simulink library "Lib_Piccolo"  (R2018b)
settings: Solver=VariableStepAuto  StartTime=0.0  StopTime=10.0  RelTol=1e-3
values from neighbouring files (symbols this model uses):
  AccelErrInt2Brakes = 0.15    [SimulationControlConfig16P.m]    (also in SimulationControlConfig16P_LEGACY.m; SimulationControlConfigTAILLESS.m = 0.2; SimulationControlConfigUTAIL.m = 0.2)
  AileronMax = 25    [SimulationControlConfig16P.m]    (also in SimulationControlConfig16P_LEGACY.m; SimulationControlConfigTAILLESS.m; SimulationControlConfigUTAIL.m)
  AileronPower = 0.00268    [SimulationControlConfig16P.m]    (also in SimulationControlConfig16P_LEGACY.m; SimulationControlConfigTAILLESS.m; SimulationControlConfigUTAIL.m)
  AileronSurfaceMax = 45    [SimulationControlConfig16P.m]    (also in SimulationControlConfig16P_LEGACY.m)
  AileronTrim = 0    [SimulationControlConfig16P.m]    (also in SimulationControlConfig16P_LEGACY.m; SimulationControlConfigTAILLESS.m; SimulationControlConfigUTAIL.m)
  Alt = 1000 + TerrainHeight    [SimulationStateConfig.m]
  AltCruise_m = testPlans(testIndx).terrainElevation * 0.3048 + 200    [SimulationControlConfig16P.m]    (also in SimulationControlConfigTAILLESS.m = 1083; SimulationControlConfigUTAIL.m = testPlans(testIndx).terrainElevation * 0.3048 + 152)
  AltitudeRate2PitchCmdIntegratorInit = 0.1    [SimulationControlPre.m]
  AltMax = 10000    [SimulationControlConfig16P.m]    (also in SimulationControlConfig16P_LEGACY.m; SimulationControlConfigTAILLESS.m; SimulationControlConfigUTAIL.m)
  AltMaxAccel = 1.25    [SimulationControlConfig16P.m]    (also in SimulationControlConfig16P_LEGACY.m = 0.9; SimulationControlConfigTAILLESS.m = 1.7; SimulationControlConfigUTAIL.m = 2)
  AltMin = 0    [SimulationControlConfig16P.m]    (also in SimulationControlConfig16P_LEGACY.m; SimulationControlConfigTAILLESS.m; SimulationControlConfigUTAIL.m)
  AltRateCmd2Pitch = 0.50    (= 0.5)    [SimulationControlConfig16P.m]    (also in SimulationControlConfig16P_LEGACY.m = 0.6; SimulationControlConfigTAILLESS.m = 0.2; SimulationControlConfigUTAIL.m = 0.3)
  AltRateError2Pitch = 0.40    (= 0.4)    [SimulationControlConfig16P.m]    (also in SimulationControlConfig16P_LEGACY.m; SimulationControlConfigTAILLESS.m = 0.55; SimulationControlConfigUTAIL.m = 0.55)
  AltRateErrorInt2Pitch = 0.50    (= 0.5)    [SimulationControlConfig16P.m]    (also in SimulationControlConfig16P_LEGACY.m = 0.45; SimulationControlConfigTAILLESS.m; SimulationControlConfigUTAIL.m = 0.75)
  AltRateLpfCutOff = 3    [SimulationControlConfig16P.m]    (also in SimulationControlConfig16P_LEGACY.m; SimulationControlConfigTAILLESS.m = 2; SimulationControlConfigUTAIL.m = 2)
  AutoNosegear2Rudder = 26    [SimulationControlConfig16P.m]    (also in SimulationControlConfig16P_LEGACY.m; SimulationControlConfigTAILLESS.m = 25.2; SimulationControlConfigUTAIL.m = 14)
  b = 5.54    [SimulationControlConfig16P.m]    (also in SimulationControlConfig16P_LEGACY.m; SimulationControlConfigTAILLESS.m = 2.37; SimulationControlConfigUTAIL.m = 2.37)
  Bank2AileronIntegratorInit = 0    [SimulationControlPre.m]
  BankMax_User = BankMax_User/180*pi    (= 0.523598775598)    [SimulationControlConfig16P.m]    (also in SimulationControlConfig16P_LEGACY.m; SimulationControlConfigTAILLESS.m = 0.610865238198; SimulationControlConfigUTAIL.m = 0.628318530718)
  baseLegFlaps = 20    [SimulationControlConfig16P.m]    (also in SimulationControlConfig16P_LEGACY.m = 0; SimulationControlConfigTAILLESS.m = 15; SimulationControlConfigUTAIL.m = 10)
  C = GeneticOpt.C    [SimulationCostFunction.m]
  c = Sw/b    (= 0.841696750903)    [SimulationControlConfig16P.m]    (also in SimulationControlConfig16P_LEGACY.m; SimulationControlConfigTAILLESS.m = 0.354008438819; SimulationControlConfigUTAIL.m = 0.354008438819)
  cell2WheelFactorMG = 5.98    [SimulationSensorConfig16P_LEGACY.m]
  cell2WheelFactorNG = 1    [SimulationSensorConfig16P_LEGACY.m]
  cellSatMaxMG = 15000    [SimulationSensorConfig16P.m]    (also in SimulationSensorConfig16P_LEGACY.m; SimulationSensorConfigTAILLESS7P.m; SimulationSensorConfigUTAIL7P.m)
  cellSatMaxNG = 1000    [SimulationSensorConfig16P.m]    (also in SimulationSensorConfig16P_LEGACY.m; SimulationSensorConfigTAILLESS7P.m; SimulationSensorConfigUTAIL7P.m)
  cellSatMinMG = -15000    [SimulationSensorConfig16P.m]    (also in SimulationSensorConfig16P_LEGACY.m; SimulationSensorConfigTAILLESS7P.m; SimulationSensorConfigUTAIL7P.m)
  cellSatMinNG = -1000    [SimulationSensorConfig16P.m]    (also in SimulationSensorConfig16P_LEGACY.m; SimulationSensorConfigTAILLESS7P.m; SimulationSensorConfigUTAIL7P.m)
  CL_Limit = CL_Max    (= 0.54)    [SimulationControlConfig16P.m]    (also in SimulationControlConfig16P_LEGACY.m; SimulationControlConfigTAILLESS.m; SimulationControlConfigUTAIL.m = 0.53)
  CL_Max = 0.54    [SimulationControlConfig16P.m]    (also in SimulationControlConfig16P_LEGACY.m; SimulationControlConfigTAILLESS.m; SimulationControlConfigUTAIL.m = 0.53)
  CL_Max_Nom = 0.465    [SimulationControlConfig16P.m]    (also in SimulationControlConfig16P_LEGACY.m; SimulationControlConfigTAILLESS.m = 0.39; SimulationControlConfigUTAIL.m)
  CL_Min = 0    [SimulationControlConfig16P.m]    (also in SimulationControlConfig16P_LEGACY.m; SimulationControlConfigTAILLESS.m; SimulationControlConfigUTAIL.m)
  ClimbMaxFraction = 0.35    [SimulationControlConfig16P.m]    (also in SimulationControlConfig16P_LEGACY.m = 0.24; SimulationControlConfigTAILLESS.m = 0.19; SimulationControlConfigUTAIL.m = 0.21)
  ClimboutMaxBank = 7.0    (= 7)    [SimulationControlConfig16P.m]    (also in SimulationControlConfig16P_LEGACY.m; SimulationControlConfigTAILLESS.m = 5; SimulationControlConfigUTAIL.m)
  ClimboutTimer = 7.0    (= 7)    [SimulationControlConfig16P.m]    (also in SimulationControlConfig16P_LEGACY.m; SimulationControlConfigTAILLESS.m; SimulationControlConfigUTAIL.m)
  dCl_per_dFlap = 0.005581818    [SimulationControlConfig16P.m]    (also in SimulationControlConfig16P_LEGACY.m = 0; SimulationControlConfigTAILLESS.m = 0; SimulationControlConfigUTAIL.m = 0)
  DecelerationCmd = 3.1    [SimulationControlConfig16P.m]    (also in SimulationControlConfig16P_LEGACY.m; SimulationControlConfigTAILLESS.m = 0.1; SimulationControlConfigUTAIL.m = 0.1)
  DeRotateLogicEndTimer = abs((NoseDownLimit_Deg-1)/DeRotateRamp_Dps)    [SimulationControlConfig16P.m]    (also in SimulationControlConfig16P_LEGACY.m; SimulationControlConfigTAILLESS.m; SimulationControlConfigUTAIL.m)
  DeRotateLogicHoldNoseUpTimer = 0.1    [SimulationControlConfig16P.m]    (also in SimulationControlConfig16P_LEGACY.m; SimulationControlConfigTAILLESS.m; SimulationControlConfigUTAIL.m)
  DeRotateLogicTimerTimeout = 2    [SimulationControlConfig16P.m]    (also in SimulationControlConfig16P_LEGACY.m; SimulationControlConfigTAILLESS.m; SimulationControlConfigUTAIL.m)
  DeRotateLowerCmdSaturation = 0    [SimulationControlConfig16P.m]    (also in SimulationControlConfig16P_LEGACY.m; SimulationControlConfigTAILLESS.m; SimulationControlConfigUTAIL.m)
  DeRotateRamp_Dps = 3    [SimulationControlConfig16P.m]    (also in SimulationControlConfig16P_LEGACY.m; SimulationControlConfigTAILLESS.m = 8; SimulationControlConfigUTAIL.m = 8)
  DeRotateUpperCmdSaturation = 7    [SimulationControlConfig16P.m]    (also in SimulationControlConfig16P_LEGACY.m; SimulationControlConfigTAILLESS.m; SimulationControlConfigUTAIL.m)
  DescentMaxFraction = 0.22    [SimulationControlConfig16P.m]    (also in SimulationControlConfig16P_LEGACY.m = 0.2; SimulationControlConfigTAILLESS.m = 0.17; SimulationControlConfigUTAIL.m = 0.17)
  DesktopSimTerrainOffset_m = 0.406    [SimulationAircraftConfig.m]
  downwindFlaps = 0    [SimulationControlConfig16P.m]    (also in SimulationControlConfig16P_LEGACY.m; SimulationControlConfigTAILLESS.m; SimulationControlConfigUTAIL.m)
  DP_init = 0.5*1.225*V_init^2    [SimulationControlConfig16P.m]    (also in SimulationControlConfig16P_LEGACY.m; SimulationControlConfigTAILLESS.m; SimulationControlConfigUTAIL.m)
  dscNoiseMG = 1    [SimulationSensorConfig16P_LEGACY.m]
  dscNoiseNG = 0.25    [SimulationSensorConfig16P_LEGACY.m]
  DSCnumBits = 24    [SimulationSensorConfig16P.m]    (also in SimulationSensorConfig16P_LEGACY.m; SimulationSensorConfigTAILLESS7P.m; SimulationSensorConfigUTAIL7P.m)
  DSCRangeMaxMG = 15000    [SimulationSensorConfig16P.m]    (also in SimulationSensorConfig16P_LEGACY.m; SimulationSensorConfigTAILLESS7P.m; SimulationSensorConfigUTAIL7P.m)
  DSCRangeMaxNG = 1000    [SimulationSensorConfig16P.m]    (also in SimulationSensorConfig16P_LEGACY.m; SimulationSensorConfigTAILLESS7P.m; SimulationSensorConfigUTAIL7P.m)
  DSCRangeMinMG = -15000    [SimulationSensorConfig16P.m]    (also in SimulationSensorConfig16P_LEGACY.m; SimulationSensorConfigTAILLESS7P.m; SimulationSensorConfigUTAIL7P.m)
  DSCRangeMinNG = -1000    [SimulationSensorConfig16P.m]    (also in SimulationSensorConfig16P_LEGACY.m; SimulationSensorConfigTAILLESS7P.m; SimulationSensorConfigUTAIL7P.m)
  dt = DLLSim.dt    [SimulationTimeStep.m]    (also in SimulationTrim.m = 0.02)
  EarlyTouchdownThreshold = 3.0    (= 3)    [SimulationControlConfig16P.m]    (also in SimulationControlConfig16P_LEGACY.m; SimulationControlConfigTAILLESS.m = 2.2; SimulationControlConfigUTAIL.m = 2.5)
  ElevatorDeflectionRate = 15    [SimulationControlConfig16P.m]    (also in SimulationControlConfig16P_LEGACY.m = 12; SimulationControlConfigTAILLESS.m = 10; SimulationControlConfigUTAIL.m = 12)
  ElevatorMax = 25    [SimulationControlConfig16P.m]    (also in SimulationControlConfig16P_LEGACY.m; SimulationControlConfigTAILLESS.m; SimulationControlConfigUTAIL.m)
  ElevatorPower = -0.002209    [SimulationControlConfig16P.m]    (also in SimulationControlConfig16P_LEGACY.m; SimulationControlConfigTAILLESS.m = -0.002956; SimulationControlConfigUTAIL.m = -0.00205983)
  ElevatorTrim = -3.5    [SimulationControlConfig16P.m]    (also in SimulationControlConfig16P_LEGACY.m; SimulationControlConfigTAILLESS.m = -6; SimulationControlConfigUTAIL.m = -8)
  elevonBias = 0    [SimulationControlConfig16P.m]    (also in SimulationControlConfig16P_LEGACY.m; SimulationControlConfigTAILLESS.m; SimulationControlConfigUTAIL.m)
  Enable_TAS_Protection = 0    [SimulationControlConfig16P.m]    (also in SimulationControlConfig16P_LEGACY.m; SimulationControlConfigTAILLESS.m; SimulationControlConfigUTAIL.m)
  EnableCrossTrackAbort = 1    [SimulationControlConfig16P.m]    (also in SimulationControlConfigTAILLESS.m; SimulationControlConfigUTAIL.m)
  EnergyBandwidth = 0.02    [SimulationControlConfig16P.m]    (also in SimulationControlConfig16P_LEGACY.m; SimulationControlConfigTAILLESS.m = 0.06; SimulationControlConfigUTAIL.m = 0.06)
  EngineLhFuelCut = 0    [SimulationAircraftConfig.m]
  EngineRhFuelCut = 0    [SimulationAircraftConfig.m]
  FastThrottleRate = 0.075    [SimulationControlConfig16P.m]    (also in SimulationControlConfig16P_LEGACY.m = 0.05; SimulationControlConfigTAILLESS.m = 0.1; SimulationControlConfigUTAIL.m = 0.1)
  FilterWarmUpTime = 2    [SimulationSensorConfig16P.m]    (also in SimulationSensorConfig16P_LEGACY.m; SimulationSensorConfigTAILLESS7P.m; SimulationSensorConfigUTAIL7P.m)
  finalApproachFlaps = 20    [SimulationControlConfig16P.m]    (also in SimulationControlConfig16P_LEGACY.m = 0; SimulationControlConfigTAILLESS.m = 22; SimulationControlConfigUTAIL.m = 10)
  FinalDescentSlope_Deg = testPlans(testIndx).descentSlope    [SimulationControlConfig16P.m]    (also in SimulationControlConfig16P_LEGACY.m; SimulationControlConfigTAILLESS.m; SimulationControlConfigUTAIL.m)
  flapMax = 0    [SimulationControlConfig16P.m]    (also in SimulationControlConfig16P_LEGACY.m; SimulationControlConfigTAILLESS.m; SimulationControlConfigUTAIL.m)
  flapRate = 7.5    [SimulationControlConfig16P.m]    (also in SimulationControlConfig16P_LEGACY.m; SimulationControlConfigTAILLESS.m = 6.6; SimulationControlConfigUTAIL.m)
  FlareHeight = 5    [SimulationControlConfig16P.m]    (also in SimulationControlConfig16P_LEGACY.m = 4.8; SimulationControlConfigTAILLESS.m = 2.5; SimulationControlConfigUTAIL.m = 2)
  FlareVerticalRate_mps = -0.4    [SimulationControlConfig16P.m]    (also in SimulationControlConfig16P_LEGACY.m = -0.5; SimulationControlConfigTAILLESS.m = -0.15; SimulationControlConfigUTAIL.m = -0.15)
  Fp_Aileron = 0.55*2*pi*RollRateLpfCutoff*dt    [SimulationControlConfig16P.m]    (also in SimulationControlConfig16P_LEGACY.m; SimulationControlConfigTAILLESS.m; SimulationControlConfigUTAIL.m)
  Fp_Alt = 0.55*AltBandwidth    (= 0.099)    [SimulationControlConfig16P.m]    (also in SimulationControlConfig16P_LEGACY.m; SimulationControlConfigTAILLESS.m = 0.587477826221; SimulationControlConfigUTAIL.m = 0.69115038379)
  Fp_AltRate = 0.55*2*pi*AltRateLpfCutOff*dt    [SimulationControlConfig16P.m]    (also in SimulationControlConfig16P_LEGACY.m; SimulationControlConfigTAILLESS.m; SimulationControlConfigUTAIL.m)
  Fp_Elevator = 0.55*2*pi*PitchRateLpfCutoff*dt    [SimulationControlConfig16P.m]    (also in SimulationControlConfig16P_LEGACY.m; SimulationControlConfigTAILLESS.m; SimulationControlConfigUTAIL.m)
  Fp_Energy = 0.55*2*pi*EnergyBandwidth    (= 0.069115038379)    [SimulationControlConfig16P.m]    (also in SimulationControlConfig16P_LEGACY.m; SimulationControlConfigTAILLESS.m = 0.207345115137; SimulationControlConfigUTAIL.m = 0.207345115137)
  Fp_Energy2 = 0.55*2*pi*EnergyBandwidth*dt    [SimulationControlConfig16P.m]    (also in SimulationControlConfig16P_LEGACY.m; SimulationControlConfigTAILLESS.m; SimulationControlConfigUTAIL.m)
  Fp_Pitch = 0.55*2*pi*PitchBandwidth    (= 2.76460153516)    [SimulationControlConfig16P.m]    (also in SimulationControlConfig16P_LEGACY.m = 3.11017672705; SimulationControlConfigTAILLESS.m = 3.80132711084; SimulationControlConfigUTAIL.m = 2.41902634326)
  Fp_Pitch_2 = 0.55*2*pi*PitchBandwidth*dt    [SimulationControlConfig16P.m]    (also in SimulationControlConfig16P_LEGACY.m; SimulationControlConfigTAILLESS.m; SimulationControlConfigUTAIL.m)
  Fp_Roll = RollBandwidth^2    (= 1)    [SimulationControlConfig16P.m]    (also in SimulationControlConfig16P_LEGACY.m = 1.44; SimulationControlConfigTAILLESS.m; SimulationControlConfigUTAIL.m)
  Fp_Rudder = 0.55*2*pi*YawRateLpfCutoff*dt    [SimulationControlConfig16P.m]    (also in SimulationControlConfig16P_LEGACY.m; SimulationControlConfigTAILLESS.m; SimulationControlConfigUTAIL.m)
  Fp_TAS = 0.55*2*pi*TASBandwidth    (= 0.103672557568)    [SimulationControlConfig16P.m]    (also in SimulationControlConfig16P_LEGACY.m; SimulationControlConfigTAILLESS.m = 0.172787595947; SimulationControlConfigUTAIL.m = 0.172787595947)
  Fp_TAS_Filter = 2*pi*TasLpfCutoff*dt    [SimulationControlConfig16P.m]    (also in SimulationControlConfig16P_LEGACY.m; SimulationControlConfigTAILLESS.m; SimulationControlConfigUTAIL.m)
  Fp_Turn = 0.55*2*pi*TurnErrLPFcutoff    (= 0.0345575191895)    [SimulationControlConfig16P.m]    (also in SimulationControlConfig16P_LEGACY.m; SimulationControlConfigTAILLESS.m = 0.172787595947; SimulationControlConfigUTAIL.m = 0.172787595947)
  Fp_TurnDerr = 0.55*2*pi*TurnDerivativeLPFcutoff    (= 0.0345575191895)    [SimulationControlConfig16P.m]    (also in SimulationControlConfig16P_LEGACY.m; SimulationControlConfigTAILLESS.m = 0.172787595947; SimulationControlConfigUTAIL.m = 0.172787595947)
  FTV = 3    [SimulationAircraftConfig.m]
  ftvStaticPositionError = 1/1.18    (= 0.847457627119)    [SimulationSensorConfig16P.m]    (also in SimulationSensorConfig16P_LEGACY.m; SimulationSensorConfigTAILLESS7P.m = 1; SimulationSensorConfigUTAIL7P.m = 1)
  g = 9.81    [SimulationStateConfig.m]
  GustSpd_Kts = testPlans(testIndx).gustSpd    [SimulationStateConfig.m]
  GustTriggerVal = testPlans(testIndx).gustTriggerVal    [SimulationStateConfig.m]
  HeadingErr2TurnRate = 0.5    [SimulationControlConfig16P.m]    (also in SimulationControlConfig16P_LEGACY.m; SimulationControlConfigTAILLESS.m; SimulationControlConfigUTAIL.m)
  HeadingErrDer2TurnRate = 0.3    [SimulationControlConfig16P.m]    (also in SimulationControlConfig16P_LEGACY.m; SimulationControlConfigTAILLESS.m; SimulationControlConfigUTAIL.m)
  IASbounce = IASstall*0.8    [SimulationControlPre.m]
  IAScruiseCMD = sqrt(2*m*9.81/(1.225*Sw*CL_cruise))    [SimulationControlConfig16P.m]    (also in SimulationControlConfig16P_LEGACY.m; SimulationControlConfigTAILLESS.m; SimulationControlConfigUTAIL.m)
  IASfinalCMD = 1.12 * IASmin    [SimulationControlConfig16P.m]    (also in SimulationControlConfig16P_LEGACY.m = 1.10 * IASmin; SimulationControlConfigTAILLESS.m = 1.10 * IASmin; SimulationControlConfigUTAIL.m = 1.15 * IASmin)
  IASflareCMD = IASstall    [SimulationControlConfig16P.m]    (also in SimulationControlConfig16P_LEGACY.m; SimulationControlConfigTAILLESS.m; SimulationControlConfigUTAIL.m)
  IASmax = 64    [SimulationControlConfig16P.m]    (also in SimulationControlConfig16P_LEGACY.m = 46; SimulationControlConfigTAILLESS.m = 38.58; SimulationControlConfigUTAIL.m = 35)
  IASmin = sqrt(2*m*9.81/(1.225*Sw*0.9*CL_Max_Nom))    [SimulationControlConfig16P.m]    (also in SimulationControlConfig16P_LEGACY.m; SimulationControlConfigTAILLESS.m; SimulationControlConfigUTAIL.m)
  IASshortCMD = IASstall    [SimulationControlConfig16P.m]    (also in SimulationControlConfig16P_LEGACY.m; SimulationControlConfigTAILLESS.m; SimulationControlConfigUTAIL.m)
  IASstall = sqrt(2*m*9.81/(1.225*Sw*CL_Max))    [SimulationControlConfig16P.m]    (also in SimulationControlConfig16P_LEGACY.m; SimulationControlConfigTAILLESS.m; SimulationControlConfigUTAIL.m)
  inFlight = 1    [SimulationControlConfig16P.m]    (also in SimulationControlConfigTAILLESS.m; SimulationControlConfigUTAIL.m)
  JetCatOffset = 5    [SimulationControlConfig16P.m]    (also in SimulationControlConfig16P_LEGACY.m)
  LaunchRollingElevator = -1.5    [SimulationControlConfig16P.m]    (also in SimulationControlConfig16P_LEGACY.m; SimulationControlConfigTAILLESS.m = 1; SimulationControlConfigUTAIL.m = 1)
  ldg_NosegearMax = 10    [SimulationControlConfig16P.m]    (also in SimulationControlConfig16P_LEGACY.m; SimulationControlConfigTAILLESS.m; SimulationControlConfigUTAIL.m)
  ldg_TrackVyErrInt2Nosegear = 0.1250    (= 0.125)    [SimulationControlConfig16P.m]    (also in SimulationControlConfig16P_LEGACY.m; SimulationControlConfigTAILLESS.m = 0.00714285714286; SimulationControlConfigUTAIL.m = 0.00714285714286)
  ldg_TrackVyErrPro2Nosegear = 0.35    [SimulationControlConfig16P.m]    (also in SimulationControlConfig16P_LEGACY.m; SimulationControlConfigTAILLESS.m = 0.0546666666667; SimulationControlConfigUTAIL.m = 0.0546666666667)
  ldg_TrackY2Vy = 0.07    [SimulationControlConfig16P.m]    (also in SimulationControlConfig16P_LEGACY.m; SimulationControlConfigTAILLESS.m = 0.17; SimulationControlConfigUTAIL.m = 0.17)
  ldg_Vy2NosegearScalingPower = 1.075    [SimulationControlConfig16P.m]    (also in SimulationControlConfig16P_LEGACY.m; SimulationControlConfigTAILLESS.m = 0.6; SimulationControlConfigUTAIL.m = 0.5)
  ldg_Y2VyScalingPower = 0.175    [SimulationControlConfig16P.m]    (also in SimulationControlConfig16P_LEGACY.m; SimulationControlConfigTAILLESS.m = 0; SimulationControlConfigUTAIL.m = 0)
  ldg_YawRate2Nosegear = 0.175    [SimulationControlConfig16P.m]    (also in SimulationControlConfig16P_LEGACY.m; SimulationControlConfigTAILLESS.m = 0.065; SimulationControlConfigUTAIL.m = 0.065)
  LiftSlope = 0.064285    [SimulationControlConfig16P.m]    (also in SimulationControlConfig16P_LEGACY.m; SimulationControlConfigTAILLESS.m = 0.058631; SimulationControlConfigUTAIL.m)
  LPFaileronInit = 0    [SimulationControlPre.m]
  LPFclestInit = 0    [SimulationControlPre.m]
  LPFenergyFFInit = 0    [SimulationControlPre.m]
  LPFtasInit = V_init + 2    [SimulationControlPre.m]
  LPFthrottleInit = ThrottleTrim    [SimulationControlPre.m]
  LPFturnErrInit = 0    [SimulationControlPre.m]
  ... (+115 more)
undefined symbols (not defined in the file or in its folder): abortFlag, alphaHPF, apmDelay, BRWNOUT, CRAWOR, CRAWUR, DiscIntNeverNeededParam, DLLSim, DLLSimStep, ECOMOR, ECOMUR, Fp_Tas, GustTrigger_HeightAgl_m, IPSTAT, LCINTEG, Ldg_Persist_Time, LOWER_FLAGS, MSG_ENABLE, NoiseStd, OLDVAL, OVERRIDE_ENABLE, OVERRIDE_VALUE, REBOOT, reversionEnable, revIASMax, revIASMin, revPitchMax, revPitchMin, revPitchRateMax, revRollMax, revRollRateMax, SAMPLE, SCALON, SensorModel, sigbuilder_block, Sim_Vx, Sim_Vy, Sim_Vz, Sim_Xpos, Sim_Ypos, Sim_Zpos, SYSOR, SYSUR, TARE, TEMPOR, TEMPUR, testIndx, testPlan, testPlans, Trim_piccoloInCmd, Trim_REFSI_FD_IN_nmodeCgShifterCmd_Ft, Trim_REFSI_FD_IN_nmodeFlapLhIBCmd_Deg, Trim_REFSI_FD_IN_nmodeFlapLhOBCmd_Deg, Trim_REFSI_FD_IN_nmodeFlapRhIBCmd_Deg, Trim_REFSI_FD_IN_nmodeFlapRhOBCmd_Deg, Trim_REFSI_FD_IN_nmodeSlatLhCmd_Deg, Trim_REFSI_FD_IN_nmodeSlatRhCmd_Deg, Trim_REFSI_FD_IN_nmodeSplrLhInbdCmd_Deg, Trim_REFSI_FD_IN_nmodeSplrLhOutbdCmd_Deg ... (+5)
libraries: simulink x866, aerolibconvert2 x60, $bdroot x52, aerolibatmos2 x5, dspswit3 x5, simulink_extras x4, dsparch4 x2, Lib_Piccolo_Alt x2, eeGeneralControl x1, dspindex x1
(part 2 of 44)

== system Lib_Piccolo/Altitude Rate to Pitch Command ==
  hdotCmd : Inport
  Feedback Bus : Inport  Port=2
  AND : Logic  IconShape=distinctive  AllPortsSameDT=off  OutDataTypeStr=boolean
  AltRateCmd2Pitch : Gain  Gain=AltRateCmd2Pitch
  AltRateError2Pitch : Gain  Gain=AltRateError2Pitch
  AltRateErrorIntegral2Pitch : Gain  Gain=AltRateErrorInt2Pitch
  Bus Selector : BusSelector  OutputSignals=hdot_m,V_mps,apMode,Pitch_Euler_rad
  Compare To Constant1 : simulink/Logic and Bit Operations/Compare To Constant  relop=<=  const=2  OutDataTypeStr=uint8
  Compare To Constant2 : simulink/Logic and Bit Operations/Compare To Constant  relop===  const=11  OutDataTypeStr=uint8
  Compare To Constant3 : simulink/Logic and Bit Operations/Compare To Constant  relop===  const=11  OutDataTypeStr=uint8
  Compare To Constant5 : simulink/Logic and Bit Operations/Compare To Constant  relop===  const=10  OutDataTypeStr=uint8
  Constant : Constant
  Constant1 : Constant  Value=0
  Constant2 : Constant  Value=AltitudeRate2PitchCmdIntegratorInit
  Constant5 : Constant  Value=FlareVerticalRate_mps
  Divide3 : Product  Inputs=*/
  Divide4 : Product  Inputs=*/
  Integrator : Subsystem
  LPF Vrate2PitchCmd : Subsystem
  Latch : Subsystem
  NOT : Logic  Operator=NOT  IconShape=distinctive  AllPortsSameDT=off  OutDataTypeStr=boolean
  NOT1 : Logic  Operator=NOT  IconShape=distinctive  AllPortsSameDT=off  OutDataTypeStr=boolean
  NOT2 : Logic  Operator=NOT  IconShape=distinctive  AllPortsSameDT=off  OutDataTypeStr=boolean
  OR : Logic  Operator=OR  IconShape=distinctive  AllPortsSameDT=off  OutDataTypeStr=boolean
  OR1 : Logic  Operator=OR  Inputs=3  IconShape=distinctive  AllPortsSameDT=off  OutDataTypeStr=boolean
  Optimisation Cost : Subsystem  Commented=on
  Rad2Deg{1..5} (5 alike) : Gain  Gain=180/pi
  "Saturation " : Saturate  UpperLimit=PitchMax  LowerLimit=PitchMin
  Sum : Sum  Inputs=|++
  Sum1 : Sum  Inputs=+-|
  Sum2 : Sum  Inputs=|++
  Sum3 : Sum  Inputs=|++
  Switch : Switch  Criteria=u2 > Threshold
  Switch1 : Switch  Threshold=10
  Switch2 : Switch  Criteria=u2 > Threshold
  Switch3 : Switch  Criteria=u2 > Threshold
  Switch4 : Switch  Threshold=4
  TASLimit : Subsystem
  Terminator{,1..4} (5 alike) : Terminator
  Triggered Subsystem : Subsystem  TreatAsAtomicUnit=on
  Unit Delay : UnitDelay  SampleTime=-1
  Unit Delay1 : UnitDelay  SampleTime=-1
  PitchCmd_Euler : Outport
  wires:
  Bus Selector/2 -> TASLimit/1(<V_mps>)  "<V_mps>"
  NOT1/1 -> Integrator/Enable
  AltRateError2Pitch/1 -> Rad2Deg3/1, Sum/2
  AltRateCmd2Pitch/1 -> Rad2Deg1/1, Sum/1
  Sum/1 -> Sum2/1
  Feedback Bus/1 -> Bus Selector/1
  Bus Selector/1 -> Sum1/2  "<hdot_m>"
  Sum1/1 -> Optimisation Cost/1(Sim.VRate Error), Divide4/1  "Sim.VRate Error"
  Rad2Deg1/1 -> Terminator/1  "AltRateCmd2Pitch"
  Rad2Deg3/1 -> Terminator1/1  "AltRateError2Pitch"
  Rad2Deg2/1 -> Terminator2/1  "AltRateErrorIntegral2Pitch"
  Divide3/1 -> AltRateCmd2Pitch/1
  Divide4/1 -> AltRateErrorIntegral2Pitch/1, AltRateError2Pitch/1  "ScaledError"
  TASLimit/1(V_mps_Limit) -> Divide4/2, Divide3/2
  LPF Vrate2PitchCmd/1(Output) -> Switch/1  "Sim_PitchCmd"
  Compare To Constant1/1 -> OR/1
  Compare To Constant2/1 -> OR/2, Triggered Subsystem/Trigger
  OR/1 -> OR1/2
  NOT/1 -> Switch/2, Switch3/2
  Bus Selector/4 -> Switch/3, LPF Vrate2PitchCmd/3(ResetValue), Switch3/3, Switch4/3  "<Pitch_Euler_rad>"
  Sum2/1 -> Sum3/1
  Rad2Deg4/1 -> Terminator4/1  "PitchOffsetBounce"
  Integrator/1(Out) -> Sum2/2, Rad2Deg2/1
  AltRateErrorIntegral2Pitch/1 -> Integrator/1(In)
  [pitchRateLimitFlag] -> Unit Delay1/1
  Unit Delay/1 -> Triggered Subsystem/1(In1)
  "Saturation "/1 -> Switch3/1
  Triggered Subsystem/1(Out1) -> Rad2Deg4/1, Sum3/2
  Compare To Constant3/1 -> Latch/1(D)
  Constant/1 -> Latch/2(Enable/!Rst)
  Compare To Constant5/1 -> AND/1
  Latch/1(Q_Latched) -> AND/2
  hdotCmd/1 -> Switch2/3
  AND/1 -> Switch2/2
  Constant5/1 -> Switch2/1
  Switch2/1 -> Divide3/1, Sum1/1
  Switch3/1 -> LPF Vrate2PitchCmd/1(Input)
  Unit Delay1/1 -> NOT1/1
  Sum3/1 -> "Saturation "/1
  OR1/1 -> LPF Vrate2PitchCmd/2(Reset), Integrator/2(Reset), NOT/1  "Reset"
  [stickMode] -> OR1/1
  Rad2Deg5/1 -> Terminator3/1  "Sim_PitchCmd"
  [ApGlobal] -> NOT2/1
  NOT2/1 -> OR1/3
  Constant1/1 -> Switch1/1
  Bus Selector/3 -> Switch4/2, Switch1/2, Compare To Constant2/1, Compare To Constant1/1, Compare To Constant5/1, Compare To Constant3/1  "<apMode>"
  Constant2/1 -> Switch4/1
  Switch1/1 -> Integrator/3(Init)
  Switch4/1 -> Switch1/3
  Switch/1 -> Unit Delay/1, Optimisation Cost/2(PitchCmd), PitchCmd_Euler/1, Rad2Deg5/1

== system Lib_Piccolo/Altitude Rate to Pitch Command LEGACY DEROTATE ==
  hdotCmd : Inport
  Feedback Bus : Inport  Port=2
  AND : Logic  IconShape=distinctive  AllPortsSameDT=off  OutDataTypeStr=boolean
  AltRateCmd2Pitch : Gain  Gain=AltRateCmd2Pitch
  AltRateError2Pitch : Gain  Gain=AltRateError2Pitch
  AltRateErrorIntegral2Pitch : Gain  Gain=AltRateErrorInt2Pitch
  Bus Selector : BusSelector  OutputSignals=hdot_m,V_mps,apMode,Pitch_Euler_rad
  Bus Selector1 : BusSelector  OutputSignals=Pitch_Euler_rad,apMode
  Compare To Constant1 : simulink/Logic and Bit Operations/Compare To Constant  relop=<=  const=2  OutDataTypeStr=uint8
  Compare To Constant2 : simulink/Logic and Bit Operations/Compare To Constant  relop===  const=11  OutDataTypeStr=uint8
  Compare To Constant3 : simulink/Logic and Bit Operations/Compare To Constant  relop===  const=11  OutDataTypeStr=uint8
  Compare To Constant4 : simulink/Logic and Bit Operations/Compare To Constant  relop=>=  const=10  OutDataTypeStr=uint8
  Compare To Constant5 : simulink/Logic and Bit Operations/Compare To Constant  relop===  const=10  OutDataTypeStr=uint8
  Constant : Constant
  Constant1 : Constant  Value=0
  Constant2 : Constant  Value=AltitudeRate2PitchCmdIntegratorInit
  Constant3 : Constant
  Constant4 : Constant  Value=0
  Constant5 : Constant  Value=FlareVerticalRate_mps
  DeRotate Logic rev 2 : Subsystem  VariantControl=DeRotateLogicRev == 2
  Divide3 : Product  Inputs=*/
  Divide4 : Product  Inputs=*/
  Integrator : Subsystem
  LPF Vrate2PitchCmd : Subsystem
  Latch : Subsystem
  Manual Switch : ManualSwitch  CurrentSetting=0
  NOT : Logic  Operator=NOT  IconShape=distinctive  AllPortsSameDT=off  OutDataTypeStr=boolean
  NOT1 : Logic  Operator=NOT  IconShape=distinctive  AllPortsSameDT=off  OutDataTypeStr=boolean
  NOT2 : Logic  Operator=NOT  IconShape=distinctive  AllPortsSameDT=off  OutDataTypeStr=boolean
  OR : Logic  Operator=OR  IconShape=distinctive  AllPortsSameDT=off  OutDataTypeStr=boolean
  Optimisation Cost : Subsystem  Commented=on
  Rad2Deg{,1..4} (5 alike) : Gain  Gain=180/pi
  "Saturation " : Saturate  UpperLimit=PitchMax  LowerLimit=PitchMin
  Sum : Sum  Inputs=|++
  Sum1 : Sum  Inputs=+-|
  Sum2 : Sum  Inputs=|++
  Sum3 : Sum  Inputs=|++
  Switch{,1..4} (5 alike) : Switch  Criteria=u2 > Threshold
  Terminator{,1..4} (5 alike) : Terminator
  Triggered Subsystem : Subsystem  TreatAsAtomicUnit=on
  Unit Delay : UnitDelay  SampleTime=-1
  Unit Delay1 : UnitDelay  SampleTime=-1
  deg2rad : Gain  Gain=pi/180
  rad2Deg : Gain  Gain=180/pi
  PitchCmd_Euler : Outport
  tag scope: DeRotateComplete=global, Sim_PitchCmd=global
  wires:
  AltRateError2Pitch/1 -> Rad2Deg3/1, Sum/2
  AltRateCmd2Pitch/1 -> Rad2Deg1/1, Sum/1
  Sum/1 -> Sum2/1
  Bus Selector/1 -> Sum1/2  "<hdot_m>"
  Sum1/1 -> Optimisation Cost/1(Sim.VRate Error), Divide4/1  "Sim.VRate Error"
  Rad2Deg1/1 -> Terminator/1  "AltRateCmd2Pitch"
  Rad2Deg3/1 -> Terminator1/1  "AltRateError2Pitch"
  Rad2Deg2/1 -> Terminator2/1  "AltRateErrorIntegral2Pitch"
  Divide3/1 -> AltRateCmd2Pitch/1
  Divide4/1 -> AltRateErrorIntegral2Pitch/1, AltRateError2Pitch/1
  Bus Selector/2 -> Divide4/2, Divide3/2  "<V_mps>"
  Constant2/1 -> Switch1/3
  Rad2Deg/1 -> Terminator3/1  "Sim.PitchCmd"
  LPF Vrate2PitchCmd/1(Output) -> Switch4/1  "Sim_PitchCmd"
  Compare To Constant1/1 -> OR/1
  Compare To Constant2/1 -> Triggered Subsystem/Trigger, OR/2
  OR/1 -> Integrator/2(Reset), NOT/1
  NOT/1 -> Switch3/2, Switch/2
  Bus Selector/3 -> Compare To Constant4/1, Compare To Constant2/1, Compare To Constant1/1, Compare To Constant5/1, Compare To Constant3/1  "<apMode>"
  Bus Selector/4 -> Switch3/3, Switch/3  "<Pitch_Euler_rad>"
  Compare To Constant4/1 -> Switch1/2
  Constant1/1 -> Switch1/1
  Sum2/1 -> Sum3/1
  Rad2Deg4/1 -> Terminator4/1  "PitchOffsetBounce"
  Integrator/1(Out) -> Sum2/2, Rad2Deg2/1
  AltRateErrorIntegral2Pitch/1 -> Integrator/1(In)
  Switch1/1 -> Integrator/3(Init)  "Sim_PitchCmd"
  [pitchRateLimitFlag] -> Unit Delay1/1
  Unit Delay/1 -> Triggered Subsystem/1(In1)
  "Saturation "/1 -> Switch3/1
  Triggered Subsystem/1(Out1) -> Sum3/2, Rad2Deg4/1
  Compare To Constant3/1 -> Latch/1(D)
  Constant/1 -> Latch/2(Enable/!Rst)
  Compare To Constant5/1 -> AND/1
  Latch/1(Q_Latched) -> AND/2
  hdotCmd/1 -> Switch2/3
  AND/1 -> Switch2/2
  Constant5/1 -> Switch2/1
  Switch2/1 -> Divide3/1, Sum1/1
  Switch3/1 -> LPF Vrate2PitchCmd/1(Input)
  Unit Delay1/1 -> NOT1/1
  NOT1/1 -> Integrator/Enable
  Sum3/1 -> "Saturation "/1
  Switch/1 -> Unit Delay/1, Optimisation Cost/2(PitchCmd), PitchCmd_Euler/1, Rad2Deg/1, [Sim_PitchCmd]  "Sim_PitchCmd"
  NOT2/1 -> Switch4/2
  rad2Deg/1 -> DeRotate Logic rev 2/1(PitchAngle_Deg)
  DeRotate Logic rev 2/1(PitchDeRotateCmd) -> deg2rad/1  "Sim_DeRotatePitchCmd_Deg"
  Constant4/1 -> DeRotate Logic rev 2/4(Pic_AssistMode)
  DeRotate Logic rev 2/3(WoWBool_Out) -> Manual Switch/1  "Sim_DeRotateComplete"
  DeRotate Logic rev 2/2(DeRotateActive) -> NOT2/1  "Sim_DeRotateCLActive"
  Feedback Bus/1 -> Bus Selector1/1, Bus Selector/1
  Bus Selector1/2 -> DeRotate Logic rev 2/2(Pic_ApMode)  "<apMode>"
  Constant3/1 -> DeRotate Logic rev 2/3(Pic_GlobalOn)
  Bus Selector1/1 -> rad2Deg/1  "<Pitch_Euler_rad>"
  Switch4/1 -> Switch/1
  deg2rad/1 -> Switch4/3
  [TouchdownDetectedFlag] -> Manual Switch/2, DeRotate Logic rev 2/5(WoWBool)
  Manual Switch/1 -> [DeRotateComplete]

== system Lib_Piccolo/Altitude Reference Model ==
  note: Need to override hdot cmd with current feedback during AP OFF to resume control from last measured value
  note: There appears to be an undocumented feedforward term Based on the Track slope
  AltCmd : Inport
  VzCmd : Inport  Port=2
  Feedback Bus : Inport  Port=3
  TAScmd : Inport  Port=4
  AND : Logic  Inputs=3  IconShape=distinctive  AllPortsSameDT=off  OutDataTypeStr=boolean
  Alt Max Accel Rate Limit : Subsystem
  Alt Saturation : Saturate  UpperLimit=AltMax  LowerLimit=AltMin
  Bus Selector : BusSelector  OutputSignals=altitude_m,V_mps,apMode,hdot_m
  ClimbFraction : Gain  Gain=ClimbMaxFraction
  Compare To Constant : simulink/Logic and Bit Operations/Compare To Constant  relop===  const=11  OutDataTypeStr=boolean
  Compare To Constant1 : simulink/Logic and Bit Operations/Compare To Constant  relop=>=  const=9  OutDataTypeStr=uint8
  Compare To Constant2 : simulink/Logic and Bit Operations/Compare To Constant  relop=>=  const=10  OutDataTypeStr=uint8
  Compare To Constant3 : simulink/Logic and Bit Operations/Compare To Constant  relop=<=  const=2  OutDataTypeStr=boolean
  Constant : Constant  Value=IASmin
  Constant1 : Constant  Value=FlareVerticalRate_mps
  Constant2 : Constant  Value=IASstall
  Constant3 : Constant  Value=IASstall
  Constant4 : Constant  Value=AltMaxAccel
  Constant5 : Constant  Value=100
  DescentFraction : Gain  Gain=-DescentMaxFraction
  Fp_Alt : Gain  Gain=Fp_Alt
  From Workspace10 : FromWorkspace  Commented=on  VariableName=REF.TrackZ  SampleTime=0
  Gain : Gain
  Gain3 : Gain  Gain=-1
  Manual Switch : ManualSwitch  CurrentSetting=0
  Max : MinMax  Function=max  Inputs=2
  NOT : Logic  Operator=NOT  IconShape=distinctive  AllPortsSameDT=off  OutDataTypeStr=boolean
  NOT1 : Logic  Operator=NOT  IconShape=distinctive  AllPortsSameDT=off  OutDataTypeStr=boolean
  OR : Logic  Operator=OR  IconShape=distinctive  AllPortsSameDT=off  OutDataTypeStr=boolean
  Saturation Dynamic : simulink/Discontinuities/Saturation Dynamic  OutMin=[]  OutMax=[]  OutDataTypeStr=Inherit: Same as second input  OutDataType=fixdt(1, 16)  OutScaling=2^-10  DoSatur=off
  Saturation Dynamic1 : simulink/Discontinuities/Saturation Dynamic  OutMin=[]  OutMax=[]  OutDataTypeStr=Inherit: Same as second input  OutDataType=fixdt(1, 16)  OutScaling=2^-10  DoSatur=off
  Sum : Sum  Inputs=|+-
  Sum1 : Sum  Inputs=|++
  Switch : Switch  Criteria=u2 > Threshold
  Switch1 : Switch  Criteria=u2 > Threshold
  Switch2 : Switch  Criteria=u2 > Threshold  Threshold=0.5
  Switch3 : Switch  Criteria=u2 > Threshold  Threshold=0.5
  VRateCmd (Alt) : Outport
  tag scope: Sim_TrackZError=global, Sim_vRateCmd=global
  wires:
  AltCmd/1 -> Alt Saturation/1
  Sum/1 -> Manual Switch/2
  DescentFraction/1 -> Saturation Dynamic/3  "Sim.DescentMaxFraction"
  ClimbFraction/1 -> Saturation Dynamic/1  "Sim.ClimbMaxFraction"
  Gain/1 -> [Sim_vRateCmd], VRateCmd (Alt)/1  "Sim.vRateCmd (Alt)"
  Alt Saturation/1 -> Sum/1
  Manual Switch/1 -> [Sim_TrackZError], Fp_Alt/1  "Sim_TrackZError"
  From Workspace10/1 -> Manual Switch/1  "REF.TrackZ"
  Bus Selector/1 -> Sum/2  "<altitude_m>"
  Saturation Dynamic1/1 -> ClimbFraction/1, DescentFraction/1
  Bus Selector/2 -> Saturation Dynamic1/2  "<V_mps>"
  Compare To Constant1/1 -> Switch/2
  Bus Selector/3 -> Compare To Constant3/1, Compare To Constant/1, Compare To Constant2/1, Compare To Constant1/1  "<apMode>"
  Constant/1 -> Switch/3
  Constant3/1 -> Switch/1
  Switch/1 -> Saturation Dynamic1/3
  Saturation Dynamic/1 -> Switch1/3
  Feedback Bus/1 -> Bus Selector/1
  Compare To Constant2/1 -> Switch1/2
  Constant1/1 -> Switch1/1
  Fp_Alt/1 -> Sum1/1
  Sum1/1 -> Saturation Dynamic/2
  Switch3/1 -> Alt Max Accel Rate Limit/2(u)
  TAScmd/1 -> Max/2
  Constant2/1 -> Max/1
  Gain3/1 -> Alt Max Accel Rate Limit/3(lo)
  Switch2/1 -> Alt Max Accel Rate Limit/1(up), Gain3/1  "altAccelLimit"
  Alt Max Accel Rate Limit/1(Y) -> Gain/1
  Max/1 -> Saturation Dynamic1/1
  VzCmd/1 -> Sum1/2
  [controllerActive] -> Switch2/2
  Constant4/1 -> Switch2/1
  Constant5/1 -> Switch2/3
  [controllerActive] -> Switch3/2
  Switch1/1 -> Switch3/1
  Bus Selector/4 -> Switch3/3  "<hdot_m>"
  AND/1 -> [controllerActive]  "Sim.VrateControllerActive"
  [ApGlobal] -> AND/2
  Compare To Constant/1 -> OR/1
  NOT/1 -> AND/3
  OR/1 -> NOT/1
  Compare To Constant3/1 -> OR/2
  NOT1/1 -> AND/1
  [stickMode] -> NOT1/1

== system Lib_Piccolo/Bank to Aileron ==
  BankCmd_Euler : Inport
  Feedback Bus : Inport  Port=2
  Bank Angle Limit Calculation : Subsystem
  Body To Euler Translation : MATLAB Function  TreatAsAtomicUnit=on
  Bus Selector : BusSelector  OutputSignals=apMode,DynamicPressure_Pa,V_mps,RollRate_Body_radps,PitchRate_Body_radps,YawRate_Body_radps,Roll_Euler_rad,Pitch_Euler_rad
  Constant : Constant  Value=RollMaxAccel
  Constant1 : Constant  Value=100
  Dynamic Inversion PID : Subsystem
  DynamicPLimit : Subsystem
  Gain : Gain  Gain=180/pi
  Gain1 : Gain  Gain=-1
  Gain2 : Gain  Gain=pi/180
  Manual Switch : ManualSwitch  CurrentSetting=0
  Reference Model : Subsystem
  Roll Rate Max Accel Rate Limit : $bdroot/Bank to Aileron/Reference Model/Roll Rate Max Accel Rate Limit  SystemSampleTime=-1
  Switch : Switch  Criteria=u2 > Threshold
  Switch1 : Switch  Criteria=u2 > Threshold
  Switch2 : Switch  Criteria=u2 > Threshold  Threshold=10
  TASLimit : Subsystem
  Aileron_Deg : Outport
  tag scope: Sim_rollRateCmd=global
  wires:
  Roll Rate Max Accel Rate Limit/1 -> Manual Switch/2, Gain/1
  Switch/1 -> Roll Rate Max Accel Rate Limit/2
  [ApGlobal] -> Switch/2
  Reference Model/1(RollRateCmd_Euler) -> Switch/1
  DynamicPLimit/1(Out1) -> Switch2/1, Bank Angle Limit Calculation/2(Q)  "Q_Lim"
  TASLimit/1(Out1) -> Dynamic Inversion PID/4(V)
  Bus Selector/3 -> TASLimit/2(<V_mps>)  "<V_mps>"
  Bus Selector/2 -> Switch2/3, DynamicPLimit/2(DynamicPressure_Pa)  "<DynamicPressure_Pa>"
  BankCmd_Euler/1 -> Reference Model/1(BankCmd_Euler)
  Manual Switch/1 -> Dynamic Inversion PID/1(RollRateCmd_Euler)
  [REFrollRateCmd] -> Gain2/1  "REF.rollRateCmdDps"
  Gain2/1 -> Manual Switch/1  "REF.rollRateCmd"
  Bus Selector/1 -> Switch2/2, Dynamic Inversion PID/5(apMode), Bank Angle Limit Calculation/1(apMode), TASLimit/1(apMode), DynamicPLimit/1(apMode)  "<apMode>"
  Dynamic Inversion PID/1(Aileron_Deg) -> Aileron_Deg/1
  Gain/1 -> [Sim_rollRateCmd]  "Sim.rollRateCmd"
  Bus Selector/8 -> Body To Euler Translation/5(Theta)  "<Pitch_Euler_rad>"
  Bus Selector/6 -> Body To Euler Translation/3(r)  "<YawRate_Body_radps>"
  Bus Selector/5 -> Body To Euler Translation/2(q)  "<PitchRate_Body_radps>"
  Bus Selector/4 -> Body To Euler Translation/1(p)  "<RollRate_Body_radps>"
  Bus Selector/7 -> Reference Model/2("Bank_Euler "), Body To Euler Translation/4(Phi)  "<Roll_Euler_rad>"
  Feedback Bus/1 -> Bus Selector/1
  Body To Euler Translation/1(PhiDot) -> Dynamic Inversion PID/2(RollRate_Euler), Switch/3
  Bank Angle Limit Calculation/1(BankMax_Euler) -> Reference Model/3("BankMax_Euler ")
  Gain1/1 -> Roll Rate Max Accel Rate Limit/3
  Switch1/1 -> Gain1/1, Roll Rate Max Accel Rate Limit/1
  [ApGlobal] -> Switch1/2
  Constant/1 -> Switch1/1
  Constant1/1 -> Switch1/3
  Switch2/1 -> Dynamic Inversion PID/3(Q)

== system Lib_Piccolo/Brake Controller ==
  Feedback Bus : Inport
  Variant Subsystem : Subsystem  Variant=on
  Brake_Pcnt : Outport
  wires:
  Feedback Bus/1 -> Variant Subsystem/1(Feedback Bus)
  Variant Subsystem/1(Brake_Pcnt) -> Brake_Pcnt/1

== system Lib_Piccolo/Control Allocation ==
  note: 1) Add Subsystem or Model blocks as valid variant choices.
      | 2) You cannot connect blocks at this level. At simulation, connectivity is automatically
      | determined, based on the active variant and port name matching.
  Aileron : Inport
  Elevator : Inport  Port=2
  Rudder : Inport  Port=3
  Throttle : Inport  Port=4
  Nosegear : Inport  Port=5
  Brake : Inport  Port=6
  Flap : Inport  Port=7
  Feedback Bus : Inport  Port=8
  M2 : Subsystem  VariantControl="ControlAllocation == \"M2\""
  "M2 Flap-to-Drag " : Subsystem  VariantControl="ControlAllocation == \"M2 FTD\""
  M2 Flaperon : Subsystem  VariantControl="ControlAllocation == \"M2 FLAPERON\""
  M2 Flaperon and FTD : Subsystem  VariantControl="ControlAllocation == \"M2 FLAPERON+\""
  M2_OLD : Subsystem  VariantControl="ControlAllocation == \"M2_OLD\""
  M7 : Subsystem  VariantControl="ControlAllocation == \"M7\""
  M8 : Subsystem  VariantControl="ControlAllocation == \"M8\""
  M8 Flap-to-Drag : Subsystem  VariantControl="ControlAllocation == \"M8 FTD\""
  "Aileron_Deg " : Outport
  "InboardElevon_Deg " : Outport  Port=2
  OutboardElevon_Deg : Outport  Port=3
  "U-TailElevator_Deg " : Outport  Port=4
  Aft-Flap_Deg : Outport  Port=5
  PylonRudder_Deg : Outport  Port=6
  WingletRudder_Deg : Outport  Port=7
  U-tailRudder_Deg : Outport  Port=8
  "Throttle_Pct " : Outport  Port=9
  Nosegear_Deg : Outport  Port=10
  Brake (0-1) : Outport  Port=11
  Flaps_Deg : Outport  Port=12
  Slats_Deg : Outport  Port=13
  Spoilers_Deg : Outport  Port=14
  Stabilizer_Deg : Outport  Port=15

== system Lib_Piccolo/Control Allocation LEGACY ==
  note: For 16.5% U-tail:
      | Aileron: aileron, inboard elevon, outboard elevon
      | Elevator: aft-flap, U-tail elevator,
      | Rudder: pylon rudder, winglet rudder, U-tail rudder
      |
      | For 16.5% Tailless (w/o U-tail elevator and U-tail rudder):
      | Aileron: aileron, inboard elevon, outboard elevon
      | Elevator: aft-flap, inboard elvon, outboard elevon
      | Rudder: pylon rudder, winglet rudder
  Aileron : Inport
  Elevator : Inport  Port=2
  Rudder : Inport  Port=3
  Throttle : Inport  Port=4
  Bus Creator : BusCreator  Inputs=6
  Constant : Constant  Value=0
  Constant1 : Constant  Value=0
  Gain{,1..7} (8 alike) : Gain
  Variant Model : Subsystem  Variant=on
  "Aileron_Deg " : Outport
  "InboardElevon_Deg " : Outport  Port=2
  OutboardElevon_Deg : Outport  Port=3
  "U-TailElevator_Deg " : Outport  Port=4
  Aft-Flap_Deg : Outport  Port=5
  PylonRudder_Deg : Outport  Port=6
  WingletRudder_Deg : Outport  Port=7
  U-tailRudder_Deg : Outport  Port=8
  "Throttle_Pct " : Outport  Port=9
  Nosegear_Deg : Outport  Port=10
  Brake (0-1) : Outport  Port=11
  tag scope: Sim_Surface=global
  wires:
  Elevator/1 -> Bus Creator/2, Gain1/1, Gain/1  "Sim_ElevatorCmd"
  Gain/1 -> "U-TailElevator_Deg "/1
  Aileron/1 -> Bus Creator/1, Gain2/1, Gain4/1, Gain3/1  "Sim_AileronCmd"
  Gain2/1 -> "Aileron_Deg "/1
  Gain3/1 -> "InboardElevon_Deg "/1
  Gain4/1 -> OutboardElevon_Deg/1
  Gain7/1 -> U-tailRudder_Deg/1
  Gain6/1 -> WingletRudder_Deg/1
  Gain5/1 -> PylonRudder_Deg/1
  Rudder/1 -> Bus Creator/3, Gain7/1, Gain6/1, Gain5/1  "Sim_RudderCmd"
  Gain1/1 -> Aft-Flap_Deg/1
  Constant/1 -> Bus Creator/5, Nosegear_Deg/1  "Sim_NosegearCmd"
  Constant1/1 -> Brake (0-1)/1, Bus Creator/6  "Sim_BrakeCmd"
  Bus Creator/1 -> [Sim_Surface]
  Throttle/1 -> Variant Model/1(Sim_ThrottleCmd), Bus Creator/4  "Sim_ThrottleCmd"
  Variant Model/1(ThrottleCmdOut) -> "Throttle_Pct "/1  "Sim_ThrottleCmd"

== system Lib_Piccolo/Cruise TAS Cmd ==
  Feedback Bus : Inport
  CAS2TAS : Subsystem
  Constant : Constant  Value=IAScruiseCMD
  Constant1 : Constant  Value=IASmax
  IAS Min Calc : $bdroot/IAS Min Calc  SystemSampleTime=-1
  Multiply : Product
  Saturation Dynamic : simulink/Discontinuities/Saturation Dynamic  OutMin=[]  OutMax=[]  OutDataTypeStr=Inherit: Same as second input  OutDataType=fixdt(1, 16)  OutScaling=2^-10  DoSatur=off
  Sim.TAScmd : Outport
  tag scope: Sim_TAScmd=global
  wires:
  CAS2TAS/1(Out1) -> Multiply/2
  Constant/1 -> Saturation Dynamic/2  "Sim.IAScmd"
  Multiply/1 -> [Sim_TAScmd], Sim.TAScmd/1  "Sim.TAScmd"
  Feedback Bus/1 -> CAS2TAS/1(In1)
  Saturation Dynamic/1 -> Multiply/1
  Constant1/1 -> Saturation Dynamic/1
  IAS Min Calc/1 -> Saturation Dynamic/3

== system Lib_Piccolo/Cruise TAS Cmd No Offset ==
  Feedback Bus : Inport
  CAS2TAS : Subsystem
  Constant : Constant  Value=IAScruiseCMD
  Constant1 : Constant  Value=IASmax
  IAS Min Calc : $bdroot/IAS Min Calc  SystemSampleTime=-1
  Multiply : Product
  Saturation Dynamic : simulink/Discontinuities/Saturation Dynamic  OutMin=[]  OutMax=[]  OutDataTypeStr=Inherit: Same as second input  OutDataType=fixdt(1, 16)  OutScaling=2^-10  DoSatur=off
  Sim.TAScmd : Outport
  tag scope: Sim_TAScmd=global
  wires:
  CAS2TAS/1(Out1) -> Multiply/2
  Constant/1 -> Saturation Dynamic/2  "Sim.IAScmd"
  Multiply/1 -> [Sim_TAScmd], Sim.TAScmd/1  "Sim.TAScmd"
  Feedback Bus/1 -> CAS2TAS/1(In1)
  Saturation Dynamic/1 -> Multiply/1
  Constant1/1 -> Saturation Dynamic/1
  IAS Min Calc/1 -> Saturation Dynamic/3

== system Lib_Piccolo/DSC Load Conversion ==
  note: NG
  note: MGL
  note: MGR
  NG_DSC_Load_N : Inport  OutDataTypeStr=single
  MGL_DSC_Load_N : Inport  Port=2  OutDataTypeStr=single
  MGR_DSC_Load_N : Inport  Port=3  OutDataTypeStr=single
  DSC-to-Wheel MGL : Subsystem
  DSC-to-Wheel MGR : Subsystem
  DSC-to-Wheel NG : Subsystem
  IsNaN : RelationalOperator  Operator=isFinite  OutDataTypeStr=boolean  RndMeth=Simplest
  IsNaN1 : RelationalOperator  Operator=isFinite  OutDataTypeStr=boolean  RndMeth=Simplest
  IsNaN2 : RelationalOperator  Operator=isFinite  OutDataTypeStr=boolean  RndMeth=Simplest
  NG_WOW_N : Outport  OutDataTypeStr=single  VectorParamsAs1DForOutWhenUnconnected=on
  NG_WOW_VALID : Outport  Port=2  OutDataTypeStr=boolean  VectorParamsAs1DForOutWhenUnconnected=on
  MGL_WOW_N : Outport  Port=3  OutDataTypeStr=single  VectorParamsAs1DForOutWhenUnconnected=on
  MGL_WOW_VALID : Outport  Port=4  OutDataTypeStr=boolean  VectorParamsAs1DForOutWhenUnconnected=on
  MGR_WOW_N : Outport  Port=5  OutDataTypeStr=single  VectorParamsAs1DForOutWhenUnconnected=on
  MGR_WOW_VALID : Outport  Port=6  OutDataTypeStr=boolean  VectorParamsAs1DForOutWhenUnconnected=on
  wires:
  NG_DSC_Load_N/1 -> DSC-to-Wheel NG/1(DSC_Load_N), IsNaN/1
  MGL_DSC_Load_N/1 -> IsNaN1/1, DSC-to-Wheel MGL/1(DSC_Load_N)
  MGR_DSC_Load_N/1 -> IsNaN2/1, DSC-to-Wheel MGR/1(DSC_Load_N)
  IsNaN/1 -> NG_WOW_VALID/1
  IsNaN1/1 -> MGL_WOW_VALID/1
  IsNaN2/1 -> MGR_WOW_VALID/1
  DSC-to-Wheel NG/1(NG_WOW_N) -> NG_WOW_N/1
  DSC-to-Wheel MGL/1(MGL_WOW_N) -> MGL_WOW_N/1
  DSC-to-Wheel MGR/1(MGR_WOW_N) -> MGR_WOW_N/1
